simulink model "initialization_test_simulink"  (R2016b)
settings: Solver=ode45  StartTime=0.0  StopTime=0.1  RelTol=1e-3
values from neighbouring files (symbols this model uses):
  ignore_inits_value = 1    [simulink_init_test.m]    (also in simulink_qp_test.m)
  pi_init = rand(nx, N)    [simulink_init_test.m]    (also in simulink_qp_test.m)
  reset_value = 1    [simulink_init_test.m]    (also in simulink_qp_test.m = 0)
  u_traj_init = rand(nu, N)    [simulink_init_test.m]    (also in simulink_qp_test.m = zeros(nu, N); test_code_reuse.m = zeros(nu, N); test_ocp_OSQP.m = zeros(nu, N); test_ocp_linear_mass_spring.m = zeros(nu, N))
  x0 = ones(nx, 1)    [create_ocp_qp_solver_formulation.m]    (also in create_ocp_solver_code_reuse.m = [0; pi; 0; 0]; create_parametric_ocp_qp.m; create_slacked_ocp_qp_solver_formulation.m; simulink_slack_test.m = [1, -3, 2])
  x_traj_init = rand(nx, N+1)    [simulink_init_test.m]    (also in simulink_qp_test.m; test_code_reuse.m = zeros(nx, N+1); test_ocp_OSQP.m = zeros(nx, N+1); test_ocp_linear_mass_spring.m = zeros(nx, N+1))
settings Model: Creator=oj  LastModifiedBy=oj
settings DataIOCC: SaveFormat=StructureWithTime  ReturnWorkspaceOutputs=on
settings OptimizationCC: LifeSpan=inf
settings DebuggingCC: FcnCallInpInsideContextMsg=warning  SFExecutionAtInitializationDiag=none
settings HardwareCC: ProdBitPerSizeT=32  ProdBitPerPtrDiffT=32  ProdWordSize=32  ProdHWDeviceType=Specified
settings ModelReferenceCC: EnableRefExpFcnMdlSchedulingChecks=off
settings SFSimCC: SimUseLocalCustomCode=on
settings RTWCC: RTWUseLocalCustomCode=on

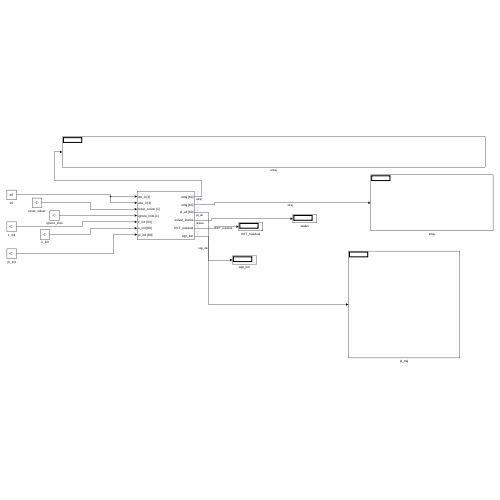
[thumbnail: Simulink's stored preview of the top-level diagram]
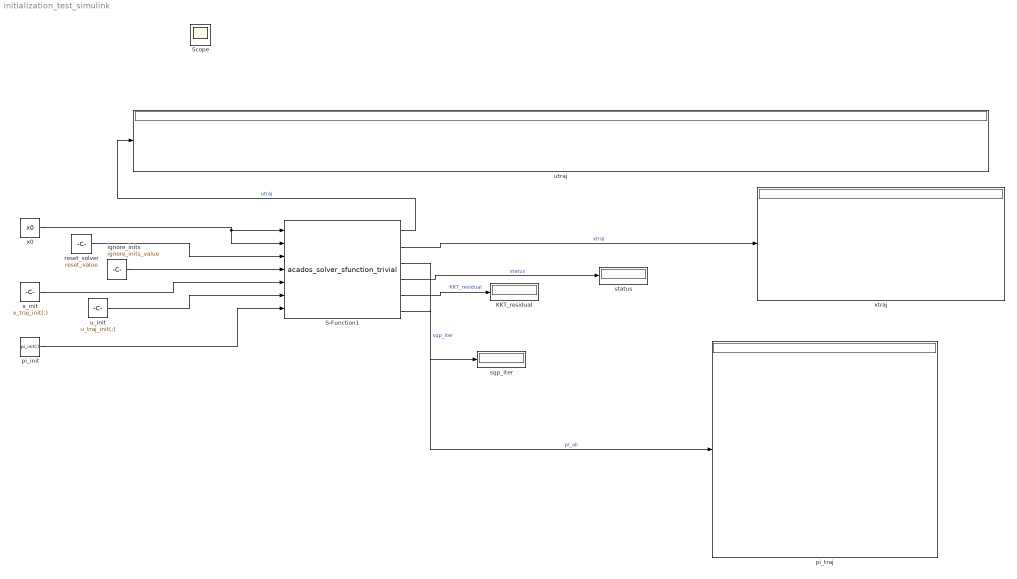
== system initialization_test_simulink ==
  KKT_residual : Display
  S-Function1 : S-Function  FunctionName=acados_solver_sfunction_trivial  SFunctionDeploymentMode=off  EnableBusSupport=off
      mask Display:
      | global sfun_input_names sfun_output_names
      | for i = 1:length(sfun_input_names)
      | 	port_label('input', i, sfun_input_names{i})
      | end
      | for i = 1:length(sfun_output_names)
      | 	port_label('output', i, sfun_output_names{i})
      | end
  ignore_inits : Constant  Value=ignore_inits_value
  pi_init : Constant  Value=pi_init(:)
  pi_traj : Display
  reset_solver : Constant  Value=reset_value
  sqp_iter : Display
  status : Display
  u_init : Constant  Value=u_traj_init(:)
  utraj : Display
  x0 : Constant  Value=x0
  x_init : Constant  Value=x_traj_init(:)
  xtraj : Display
  Scope : Scope
  wires:
  S-Function1/5 -> KKT_residual/1  "KKT_residual"
  S-Function1/1 -> utraj/1  "utraj"
  x0/1 -> S-Function1/2, S-Function1/1
  S-Function1/2 -> xtraj/1  "xtraj"
  u_init/1 -> S-Function1/6
  pi_init/1 -> S-Function1/7
  S-Function1/6 -> sqp_iter/1  "sqp_iter"
  S-Function1/4 -> status/1  "status"
  S-Function1/3 -> pi_traj/1  "pi_all"
  x_init/1 -> S-Function1/5
  reset_solver/1 -> S-Function1/3
  ignore_inits/1 -> S-Function1/4
